simulink model "motor_2gdl"  (R2026a)
settings: Solver=ode45  StopTime=2  MaxStep=1e-3
settings Model: Creator=juand  LastModifiedBy=juand

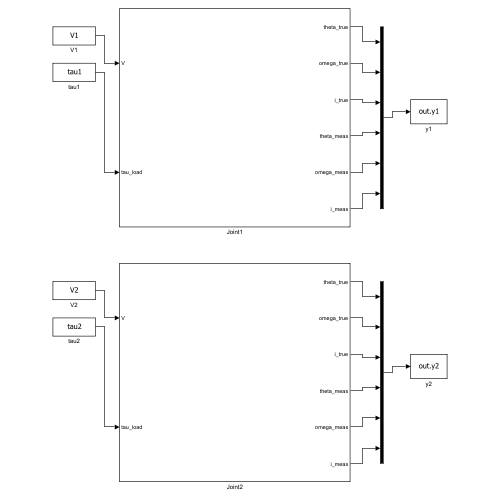
[thumbnail: Simulink's stored preview of the top-level diagram]
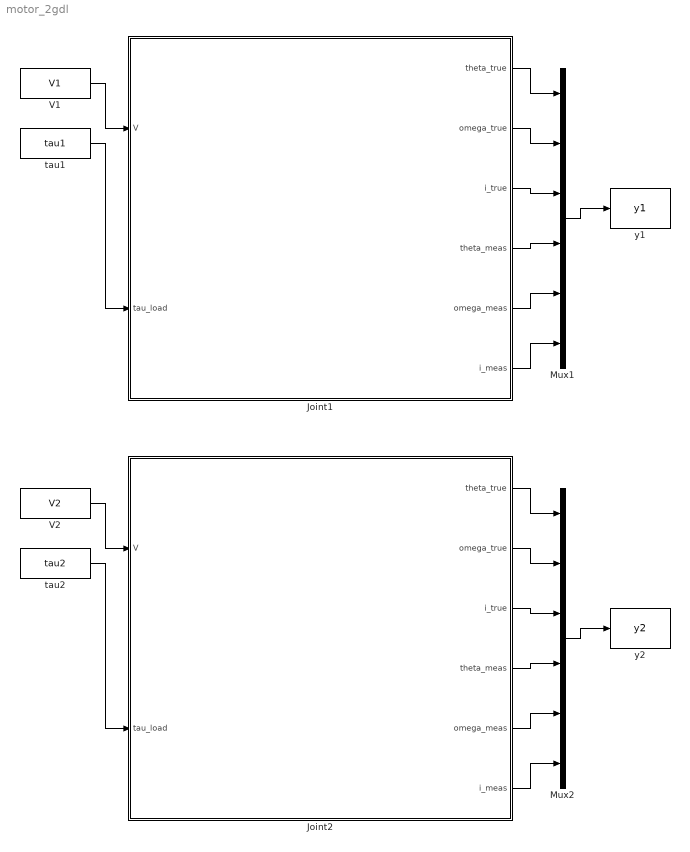
== system motor_2gdl ==
  Joint1 : Subsystem
  Joint2 : Subsystem
  Mux1 : Mux  Inputs=6
  Mux2 : Mux  Inputs=6
  V1 : FromWorkspace  VariableName=V1  OutputAfterFinalValue=Holding final value
  V2 : FromWorkspace  VariableName=V2  OutputAfterFinalValue=Holding final value
  tau1 : FromWorkspace  VariableName=tau1  OutputAfterFinalValue=Holding final value
  tau2 : FromWorkspace  VariableName=tau2  OutputAfterFinalValue=Holding final value
  y1 : ToWorkspace  VariableName=y1  SaveFormat=Timeseries  SampleTime=-1
  y2 : ToWorkspace  VariableName=y2  SaveFormat=Timeseries  SampleTime=-1
  wires:
  V1/1 -> Joint1/1(V)
  tau1/1 -> Joint1/2(tau_load)
  V2/1 -> Joint2/1(V)
  tau2/1 -> Joint2/2(tau_load)
  Joint1/1(theta_true) -> Mux1/1
  Joint2/1(theta_true) -> Mux2/1
  Joint1/2(omega_true) -> Mux1/2
  Joint2/2(omega_true) -> Mux2/2
  Joint1/3(i_true) -> Mux1/3
  Joint2/3(i_true) -> Mux2/3
  Joint1/4(theta_meas) -> Mux1/4
  Joint2/4(theta_meas) -> Mux2/4
  Joint1/5(omega_meas) -> Mux1/5
  Joint2/5(omega_meas) -> Mux2/5
  Joint1/6(i_meas) -> Mux1/6
  Joint2/6(i_meas) -> Mux2/6
  Mux1/1 -> y1/1
  Mux2/1 -> y2/1

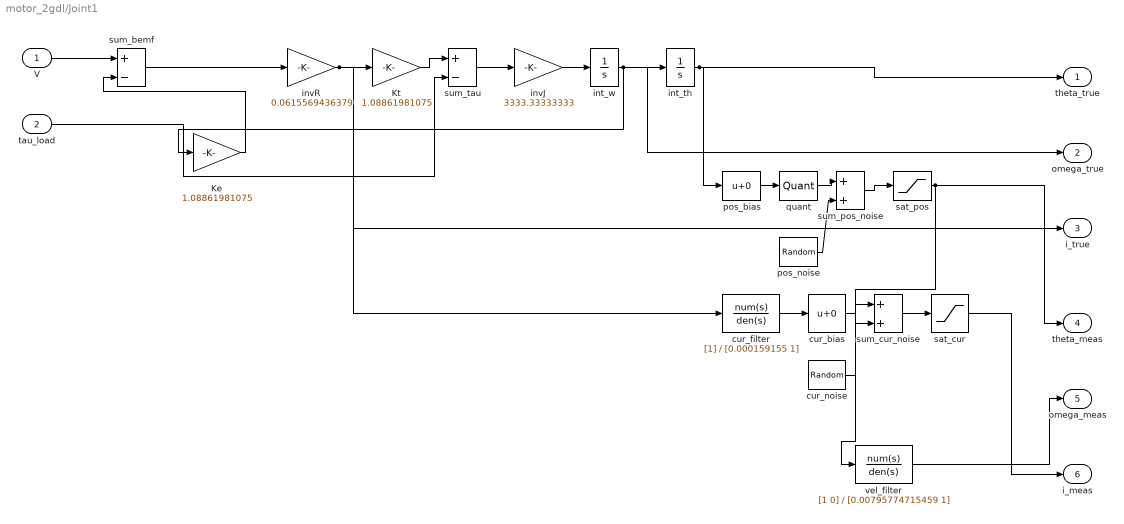
== system motor_2gdl/Joint1 ==
  V : Inport
  tau_load : Inport  Port=2
  Ke : Gain  Gain=1.08861981075
  Kt : Gain  Gain=1.08861981075
  cur_bias : Bias  SaturateOnIntegerOverflow=off
  cur_filter : TransferFcn  Denominator=[0.000159155 1]
  cur_noise : RandomNumber  Variance=4e-06  Seed=12346  SampleTime=0.01
  int_th : Integrator
  int_w : Integrator
  invJ : Gain  Gain=3333.33333333
  invR : Gain  Gain=0.0615569436379
  pos_bias : Bias  SaturateOnIntegerOverflow=off
  pos_noise : RandomNumber  Variance=7.61543549467e-07  Seed=12345  SampleTime=0.01
  quant : Quantizer  QuantizationInterval=0.00872664625997
  sat_cur : Saturate  UpperLimit=1  LowerLimit=-1
  sat_pos : Saturate  UpperLimit=1.57079632679  LowerLimit=-1.57079632679
  sum_bemf : Sum  Inputs=+-
  sum_cur_noise : Sum
  sum_pos_noise : Sum
  sum_tau : Sum  Inputs=+-
  vel_filter : TransferFcn  Numerator=[1 0]  Denominator=[0.00795774715459 1]
  theta_true : Outport
  omega_true : Outport  Port=2
  i_true : Outport  Port=3
  theta_meas : Outport  Port=4
  omega_meas : Outport  Port=5
  i_meas : Outport  Port=6
  wires:
  ? -> ?
  V/1 -> sum_bemf/1
  Ke/1 -> sum_bemf/2
  sum_bemf/1 -> invR/1
  invR/1 -> Kt/1, i_true/1, cur_filter/1
  Kt/1 -> sum_tau/1
  tau_load/1 -> sum_tau/2
  sum_tau/1 -> invJ/1
  invJ/1 -> int_w/1
  int_w/1 -> int_th/1, Ke/1, omega_true/1
  int_th/1 -> theta_true/1, pos_bias/1
  pos_bias/1 -> quant/1
  quant/1 -> sum_pos_noise/1
  pos_noise/1 -> sum_pos_noise/2
  sum_pos_noise/1 -> sat_pos/1
  sat_pos/1 -> theta_meas/1, vel_filter/1
  cur_filter/1 -> cur_bias/1
  cur_bias/1 -> sum_cur_noise/1
  cur_noise/1 -> sum_cur_noise/2
  sum_cur_noise/1 -> sat_cur/1
  sat_cur/1 -> i_meas/1
  vel_filter/1 -> omega_meas/1

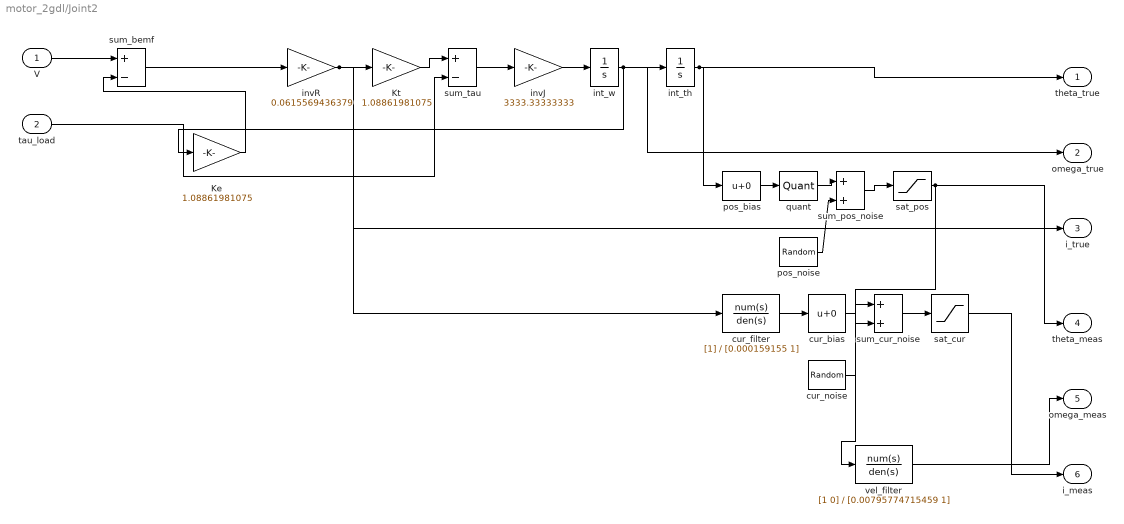
== system motor_2gdl/Joint2 ==
  V : Inport
  tau_load : Inport  Port=2
  Ke : Gain  Gain=1.08861981075
  Kt : Gain  Gain=1.08861981075
  cur_bias : Bias  SaturateOnIntegerOverflow=off
  cur_filter : TransferFcn  Denominator=[0.000159155 1]
  cur_noise : RandomNumber  Variance=4e-06  Seed=67891  SampleTime=0.01
  int_th : Integrator
  int_w : Integrator
  invJ : Gain  Gain=3333.33333333
  invR : Gain  Gain=0.0615569436379
  pos_bias : Bias  SaturateOnIntegerOverflow=off
  pos_noise : RandomNumber  Variance=7.61543549467e-07  Seed=67890  SampleTime=0.01
  quant : Quantizer  QuantizationInterval=0.00872664625997
  sat_cur : Saturate  UpperLimit=1  LowerLimit=-1
  sat_pos : Saturate  UpperLimit=1.57079632679  LowerLimit=-1.57079632679
  sum_bemf : Sum  Inputs=+-
  sum_cur_noise : Sum
  sum_pos_noise : Sum
  sum_tau : Sum  Inputs=+-
  vel_filter : TransferFcn  Numerator=[1 0]  Denominator=[0.00795774715459 1]
  theta_true : Outport
  omega_true : Outport  Port=2
  i_true : Outport  Port=3
  theta_meas : Outport  Port=4
  omega_meas : Outport  Port=5
  i_meas : Outport  Port=6
  wires:
  ? -> ?
  V/1 -> sum_bemf/1
  Ke/1 -> sum_bemf/2
  sum_bemf/1 -> invR/1
  invR/1 -> Kt/1, i_true/1, cur_filter/1
  Kt/1 -> sum_tau/1
  tau_load/1 -> sum_tau/2
  sum_tau/1 -> invJ/1
  invJ/1 -> int_w/1
  int_w/1 -> int_th/1, Ke/1, omega_true/1
  int_th/1 -> theta_true/1, pos_bias/1
  pos_bias/1 -> quant/1
  quant/1 -> sum_pos_noise/1
  pos_noise/1 -> sum_pos_noise/2
  sum_pos_noise/1 -> sat_pos/1
  sat_pos/1 -> theta_meas/1, vel_filter/1
  cur_filter/1 -> cur_bias/1
  cur_bias/1 -> sum_cur_noise/1
  cur_noise/1 -> sum_cur_noise/2
  sum_cur_noise/1 -> sat_cur/1
  sat_cur/1 -> i_meas/1
  vel_filter/1 -> omega_meas/1
